simulink library "Tire_Utilities"  (R2026a)
settings: Solver=VariableStepAuto
undefined symbols (not defined in the file or in its folder): X, Y, Z
libraries: simulink x12, nesl_utility x7, sm_lib x7, $bdroot x6
Description:
  | Simscape Vehicle Templates Library
  | 
  | Copyright 2018-2024 The MathWorks, Inc.
settings Model: Creator=smiller  LastModifiedBy=andrei

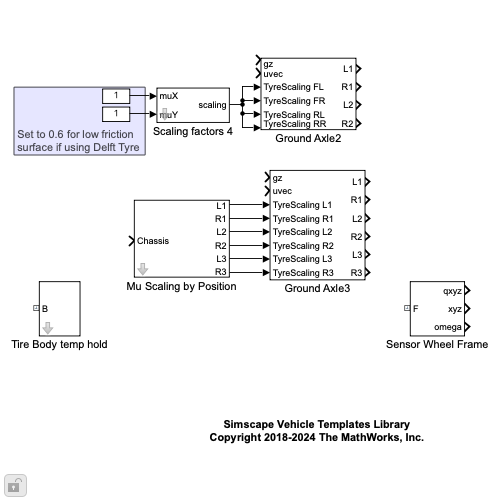
[thumbnail: Simulink's stored preview of the top-level diagram]
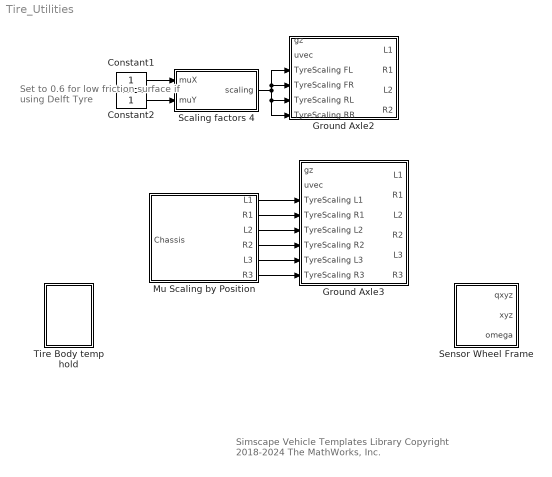
== system Tire_Utilities ==
  note: Set to 0.6 for low friction
      | surface if using Delft Tyre
  note: Simscape Vehicle Templates Library
      | Copyright 2018-2024 The MathWorks, Inc.
  Constant1 : Constant
  Constant2 : Constant
  Ground Axle2 : Subsystem
  Ground Axle3 : Subsystem
  Mu Scaling by Position : Subsystem  mask{muFL_out=1, muFR_out=1, muRL_out=1, muRR_out=1, muFL_in=1, muFR_in=1, muRL_in=1, muRR_in=1, intvX_FL_start=100-40, intvX_FR_start=100-40, intvX_RL_start=100-40, intvX_RR_start=100-40, intvX_FL_end=130-40, intvX_FR_end=130-40, intvX_RL_end=130-40, intvX_RR_end=130-40, intvY_FL_start=-30, intvY_FR_start=-30, intvY_RL_start=-30, intvY_RR_start=-30, intvY_FL_end=0, intvY_FR_end=0, intvY_RL_end=0, intvY_RR_end=0}
      mask TypeOptions muFL_out: muL1 out/Value
      mask TypeOptions muFR_out: muR1 out/Value
      mask TypeOptions muRL_out: muL2 out/Value
      mask TypeOptions muRR_out: muR2 out/Value
      mask TypeOptions muFL_in: muL 1in/Value
      mask TypeOptions muFR_in: muR1 in/Value
      mask TypeOptions muRL_in: muL2 in/Value
      mask TypeOptions muRR_in: muR2 in/Value
      mask TypeOptions intvX_FL_start: Interval Test L1x/lowlimit
      mask TypeOptions intvX_FR_start: Interval Test R1x/lowlimit
      mask TypeOptions intvX_RL_start: Interval Test L2x/lowlimit
      mask TypeOptions intvX_RR_start: Interval Test R2x/lowlimit
      mask TypeOptions intvX_FL_end: Interval Test L1x/uplimit
      mask TypeOptions intvX_FR_end: Interval Test R1x/uplimit
      mask TypeOptions intvX_RL_end: Interval Test L2x/uplimit
      mask TypeOptions intvX_RR_end: Interval Test R2x/uplimit
      mask TypeOptions intvY_FL_start: Interval Test L1y/lowlimit
      mask TypeOptions intvY_FR_start: Interval Test R1y/lowlimit
      mask TypeOptions intvY_RL_start: Interval Test L2y/lowlimit
      mask TypeOptions intvY_RR_start: Interval Test R2y/lowlimit
      mask TypeOptions intvY_FL_end: Interval Test L1y/uplimit
      mask TypeOptions intvY_FR_end: Interval Test R1y/uplimit
      mask TypeOptions intvY_RL_end: Interval Test L2y/uplimit
      mask TypeOptions intvY_RR_end: Interval Test R2y/uplimit
      mask DialogControl text_whl Prompt: Wheel
      mask DialogControl text_FL Prompt: FL
      mask DialogControl text_FR Prompt: FR
      mask DialogControl text_RL Prompt: RL
      mask DialogControl text_RR Prompt: RR
      mask DialogControl text_mu Prompt: mu
      mask DialogControl text_mu_intv Prompt: mu intv
      mask DialogControl text_x_start Prompt: X Start (m)
      mask DialogControl text_x_end Prompt: X End (m)
      mask DialogControl text_y_start Prompt: Y Start (m)
      mask DialogControl text_y_end Prompt: Y End (m)
  Scaling factors 4 : Subsystem  mask{LKX=1, LKY=1, LKYC=1, LTR=1, LKZC=1}
      mask prompts: LKX "longitudinal slip stiffness"; LKY "cornering stiffness"; LKYC "camber stiffness"; LTR "pneumatic trail"; LKZC "camber torque stiffness"
  Sensor Wheel Frame : Subsystem
  Tire Body temp hold : Subsystem  mask{radius=0.4225, rim_radius=0.3048, width=0.235, rim_width=0.235*0.1, mass=10, rim_mass=0, tire_inertia=[1 2], rim_inertia=[0 0], popup_leftRight=Left, clr_tyre=[0.5 0.5 0.5], opc_tyre=1.0, clr_rim=[0.8 0.8 0.8], opc_rim=0.5}
      mask prompts: popup_leftRight "Left/Right"
      mask init:
      | % Change rim location if wheel is on right side
      | if (popup_leftRight == 1)
      |     rhs_tire = 1;
      | elseif(popup_leftRight == 2)
      |     rhs_tire = -1;
      | end
      | 
      | Imat = [tire_inertia(1)+rim_inertia(1) 0 0; 0 tire_inertia(1)+rim_inertia(1) 0; 0 0 tire_inertia(2)+rim_inertia(2)];
      mask TypeOptions popup_leftRight: Left | Right
      mask TypeOptions clr_tyre: Tire/GraphicDiffuseColor
      mask TypeOptions opc_tyre: Tire/GraphicOpacity
      mask TypeOptions clr_rim: Rim/GraphicDiffuseColor
      mask TypeOptions opc_rim: Rim/GraphicOpacity
      mask DialogControl cont_tyre Prompt: Tire Geometry
      mask DialogControl group_tyre_dim Prompt: Dimensions
      mask DialogControl text_tyre_tire Prompt: Tyre
      mask DialogControl text_tyre_rim Prompt: Rim
      mask DialogControl text_tyre_dim_radius Prompt: Radius (m)
      mask DialogControl text_tyre_dim_width Prompt: Width (m)
      mask DialogControl text_tyre_mass Prompt: Mass (kg)
      mask DialogControl text_tyre_inertia Prompt: Inertia [Ixx Iyy]
      mask DialogControl cont_tyre_vis Prompt: Visualization
      mask DialogControl text_vis_tyre_clr Prompt: Color [RGB]
      mask DialogControl text_vis_tyre_opc Prompt: Opacity (0-1)
      mask DialogControl text_vis_tyre_tyre Prompt: Tyre
      mask DialogControl text_vis_tyre_rim Prompt: Rim
  wires:
  Mu Scaling by Position/6(R3) -> Ground Axle3/8(TyreScaling R3)
  Mu Scaling by Position/5(L3) -> Ground Axle3/7(TyreScaling L3)
  Mu Scaling by Position/4(R2) -> Ground Axle3/6(TyreScaling R2)
  Mu Scaling by Position/3(L2) -> Ground Axle3/5(TyreScaling L2)
  Mu Scaling by Position/2(R1) -> Ground Axle3/4(TyreScaling R1)
  Mu Scaling by Position/1(L1) -> Ground Axle3/3(TyreScaling L1)
  Constant2/1 -> Scaling factors 4/2(muY)
  Constant1/1 -> Scaling factors 4/1(muX)
  Scaling factors 4/1(scaling) -> Ground Axle2/4(TyreScaling FR), Ground Axle2/3(TyreScaling FL), Ground Axle2/5(TyreScaling RL), Ground Axle2/6(TyreScaling RR)

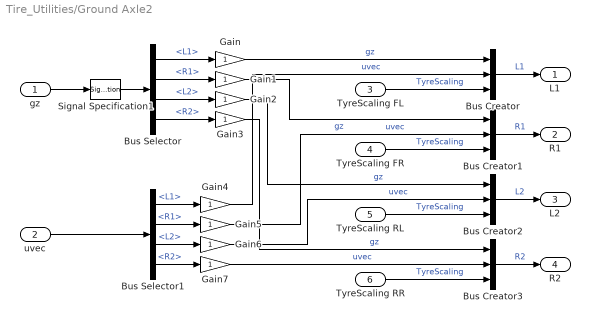
== system Tire_Utilities/Ground Axle2 ==
  gz : Inport
  uvec : Inport  Port=2
  TyreScaling FL : Inport  Port=3
  TyreScaling FR : Inport  Port=4
  TyreScaling RL : Inport  Port=5
  TyreScaling RR : Inport  Port=6
  Bus Creator{,1..3} (4 alike) : BusCreator  Inputs=3
  Bus Selector : BusSelector  OutputSignals=L1,R1,L2,R2
  Bus Selector1 : BusSelector  OutputSignals=L1,R1,L2,R2
  Gain{,1..7} (8 alike) : Gain
  Signal Specification1 : SignalSpecification  Unit=m
  L1 : Outport  VectorParamsAs1DForOutWhenUnconnected=off
  R1 : Outport  Port=2  VectorParamsAs1DForOutWhenUnconnected=off
  L2 : Outport  Port=3  VectorParamsAs1DForOutWhenUnconnected=off
  R2 : Outport  Port=4  VectorParamsAs1DForOutWhenUnconnected=off
  wires:
  Gain7/1 -> Bus Creator3/2  "uvec"
  Gain6/1 -> Bus Creator2/2  "uvec"
  Gain5/1 -> Bus Creator1/2  "uvec"
  Gain4/1 -> Bus Creator/2  "uvec"
  Bus Selector1/4 -> Gain7/1  "<R2>"
  Bus Selector1/3 -> Gain6/1  "<L2>"
  Bus Selector1/2 -> Gain5/1  "<R1>"
  Bus Selector1/1 -> Gain4/1  "<L1>"
  uvec/1 -> Bus Selector1/1
  Bus Selector/4 -> Gain3/1  "<R2>"
  Bus Selector/3 -> Gain2/1  "<L2>"
  Bus Selector/2 -> Gain1/1  "<R1>"
  Gain/1 -> Bus Creator/1  "gz"
  Bus Selector/1 -> Gain/1  "<L1>"
  TyreScaling RR/1 -> Bus Creator3/3  "TyreScaling"
  TyreScaling RL/1 -> Bus Creator2/3  "TyreScaling"
  TyreScaling FR/1 -> Bus Creator1/3  "TyreScaling"
  Gain2/1 -> Bus Creator2/1  "gz"
  Signal Specification1/1 -> Bus Selector/1
  Bus Creator2/1 -> L2/1  "L2"
  Gain3/1 -> Bus Creator3/1  "gz"
  gz/1 -> Signal Specification1/1
  Bus Creator3/1 -> R2/1  "R2"
  TyreScaling FL/1 -> Bus Creator/3  "TyreScaling"
  Gain1/1 -> Bus Creator1/1  "gz"
  Bus Creator1/1 -> R1/1  "R1"
  Bus Creator/1 -> L1/1  "L1"

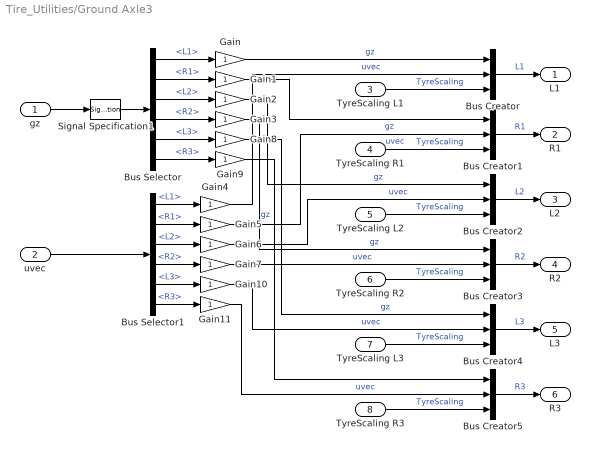
== system Tire_Utilities/Ground Axle3 ==
  gz : Inport
  uvec : Inport  Port=2
  TyreScaling L1 : Inport  Port=3
  TyreScaling R1 : Inport  Port=4
  TyreScaling L2 : Inport  Port=5
  TyreScaling R2 : Inport  Port=6
  TyreScaling L3 : Inport  Port=7
  TyreScaling R3 : Inport  Port=8
  Bus Creator{,1..5} (6 alike) : BusCreator  Inputs=3
  Bus Selector : BusSelector  OutputSignals=L1,R1,L2,R2,L3,R3
  Bus Selector1 : BusSelector  OutputSignals=L1,R1,L2,R2,L3,R3
  Gain{,1..11} (12 alike) : Gain
  Signal Specification1 : SignalSpecification  Unit=m
  L1 : Outport  VectorParamsAs1DForOutWhenUnconnected=off
  R1 : Outport  Port=2  VectorParamsAs1DForOutWhenUnconnected=off
  L2 : Outport  Port=3  VectorParamsAs1DForOutWhenUnconnected=off
  R2 : Outport  Port=4  VectorParamsAs1DForOutWhenUnconnected=off
  L3 : Outport  Port=5  VectorParamsAs1DForOutWhenUnconnected=off
  R3 : Outport  Port=6  VectorParamsAs1DForOutWhenUnconnected=off
  wires:
  Bus Selector/6 -> Gain9/1  "<R3>"
  Bus Selector/5 -> Gain8/1  "<L3>"
  Bus Selector1/6 -> Gain11/1  "<R3>"
  Bus Selector1/5 -> Gain10/1  "<L3>"
  Gain11/1 -> Bus Creator5/2  "uvec"
  Gain10/1 -> Bus Creator4/2  "uvec"
  TyreScaling R3/1 -> Bus Creator5/3  "TyreScaling"
  TyreScaling L3/1 -> Bus Creator4/3  "TyreScaling"
  Gain8/1 -> Bus Creator4/1  "gz"
  Bus Creator4/1 -> L3/1  "L3"
  Gain9/1 -> Bus Creator5/1  "gz"
  Bus Creator5/1 -> R3/1  "R3"
  Bus Creator/1 -> L1/1  "L1"
  Bus Creator1/1 -> R1/1  "R1"
  Gain1/1 -> Bus Creator1/1  "gz"
  TyreScaling L1/1 -> Bus Creator/3  "TyreScaling"
  Bus Creator3/1 -> R2/1  "R2"
  gz/1 -> Signal Specification1/1
  Gain3/1 -> Bus Creator3/1  "gz"
  Bus Creator2/1 -> L2/1  "L2"
  Signal Specification1/1 -> Bus Selector/1
  Gain2/1 -> Bus Creator2/1  "gz"
  TyreScaling R1/1 -> Bus Creator1/3  "TyreScaling"
  TyreScaling L2/1 -> Bus Creator2/3  "TyreScaling"
  TyreScaling R2/1 -> Bus Creator3/3  "TyreScaling"
  Bus Selector/1 -> Gain/1  "<L1>"
  Gain/1 -> Bus Creator/1  "gz"
  Bus Selector/2 -> Gain1/1  "<R1>"
  Bus Selector/3 -> Gain2/1  "<L2>"
  Bus Selector/4 -> Gain3/1  "<R2>"
  uvec/1 -> Bus Selector1/1
  Bus Selector1/1 -> Gain4/1  "<L1>"
  Bus Selector1/2 -> Gain5/1  "<R1>"
  Bus Selector1/3 -> Gain6/1  "<L2>"
  Bus Selector1/4 -> Gain7/1  "<R2>"
  Gain4/1 -> Bus Creator/2  "uvec"
  Gain5/1 -> Bus Creator1/2  "uvec"
  Gain6/1 -> Bus Creator2/2  "uvec"
  Gain7/1 -> Bus Creator3/2  "uvec"

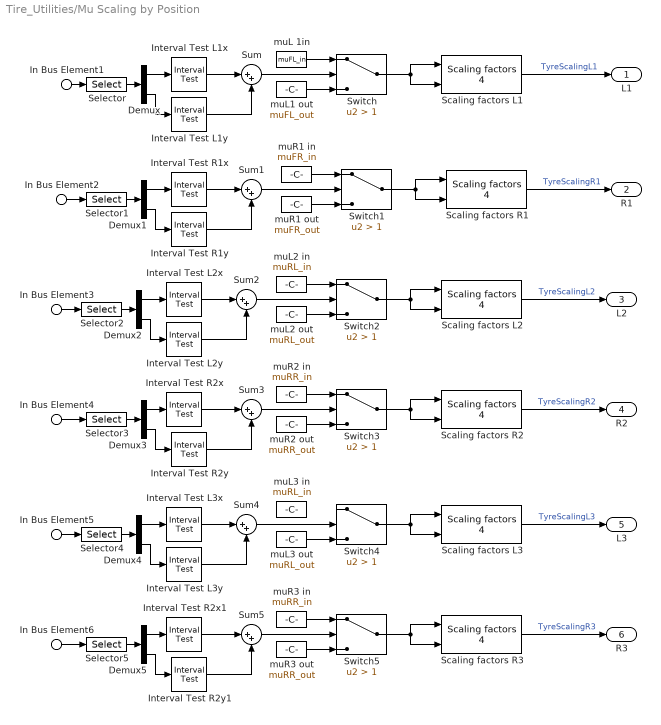
== system Tire_Utilities/Mu Scaling by Position ==
  In Bus Element1 : Inport  PortName=Chassis  Element=WhlL1.xyz
  In Bus Element2 : Inport  PortName=Chassis  Element=WhlR1.xyz
  In Bus Element3 : Inport  PortName=Chassis  Element=WhlL2.xyz
  In Bus Element4 : Inport  PortName=Chassis  Element=WhlR2.xyz
  In Bus Element5 : Inport  PortName=Chassis  Element=WhlL3.xyz
  In Bus Element6 : Inport  PortName=Chassis  Element=WhlR3.xyz
  Demux{,1..5} (6 alike) : Demux  Outputs=2
  Interval Test L1x : simulink/Logic and Bit Operations/Interval Test  IntervalClosedRight=on  uplimit=intvX_FL_end  IntervalClosedLeft=on  lowlimit=intvX_FL_start  OutDataTypeStr=uint8
  Interval Test L1y : simulink/Logic and Bit Operations/Interval Test  IntervalClosedRight=on  uplimit=intvY_FL_end  IntervalClosedLeft=on  lowlimit=intvY_FL_start  OutDataTypeStr=uint8
  Interval Test L2x : simulink/Logic and Bit Operations/Interval Test  IntervalClosedRight=on  uplimit=intvX_RL_end  IntervalClosedLeft=on  lowlimit=intvX_RL_start  OutDataTypeStr=uint8
  Interval Test L2y : simulink/Logic and Bit Operations/Interval Test  IntervalClosedRight=on  uplimit=intvY_RL_end  IntervalClosedLeft=on  lowlimit=intvY_RL_start  OutDataTypeStr=uint8
  Interval Test L3x : simulink/Logic and Bit Operations/Interval Test  IntervalClosedRight=on  uplimit=intvX_RL_end  IntervalClosedLeft=on  lowlimit=intvX_RL_start  OutDataTypeStr=uint8
  Interval Test L3y : simulink/Logic and Bit Operations/Interval Test  IntervalClosedRight=on  uplimit=intvY_RL_end  IntervalClosedLeft=on  lowlimit=intvY_RL_start  OutDataTypeStr=uint8
  Interval Test R1x : simulink/Logic and Bit Operations/Interval Test  IntervalClosedRight=on  uplimit=intvX_FR_end  IntervalClosedLeft=on  lowlimit=intvX_FR_start  OutDataTypeStr=uint8
  Interval Test R1y : simulink/Logic and Bit Operations/Interval Test  IntervalClosedRight=on  uplimit=intvY_FR_end  IntervalClosedLeft=on  lowlimit=intvY_FR_start  OutDataTypeStr=uint8
  Interval Test R2x : simulink/Logic and Bit Operations/Interval Test  IntervalClosedRight=on  uplimit=intvX_RR_end  IntervalClosedLeft=on  lowlimit=intvX_RR_start  OutDataTypeStr=uint8
  Interval Test R2x1 : simulink/Logic and Bit Operations/Interval Test  IntervalClosedRight=on  uplimit=intvX_RR_end  IntervalClosedLeft=on  lowlimit=intvX_RR_start  OutDataTypeStr=uint8
  Interval Test R2y : simulink/Logic and Bit Operations/Interval Test  IntervalClosedRight=on  uplimit=intvY_RR_end  IntervalClosedLeft=on  lowlimit=intvY_RR_start  OutDataTypeStr=uint8
  Interval Test R2y1 : simulink/Logic and Bit Operations/Interval Test  IntervalClosedRight=on  uplimit=intvY_RR_end  IntervalClosedLeft=on  lowlimit=intvY_RR_start  OutDataTypeStr=uint8
  Scaling factors L1 : $bdroot/Scaling factors 4  LKX=1  LKY=1  LKYC=1  LTR=1  LKZC=1
  Scaling factors L2 : $bdroot/Scaling factors 4  LKX=1  LKY=1  LKYC=1  LTR=1  LKZC=1
  Scaling factors L3 : $bdroot/Scaling factors 4  LKX=1  LKY=1  LKYC=1  LTR=1  LKZC=1
  Scaling factors R1 : $bdroot/Scaling factors 4  LKX=1  LKY=1  LKYC=1  LTR=1  LKZC=1
  Scaling factors R2 : $bdroot/Scaling factors 4  LKX=1  LKY=1  LKYC=1  LTR=1  LKZC=1
  Scaling factors R3 : $bdroot/Scaling factors 4  LKX=1  LKY=1  LKYC=1  LTR=1  LKZC=1
  Selector{,1..5} (6 alike) : Selector  InputPortWidth=3  IndexOptions=Index vector (dialog)  Indices=[1 2]  OutputSizes=1
  Sum{,1..5} (6 alike) : Sum  Inputs=|++
  Switch : Switch  Criteria=u2 > Threshold  Threshold=1  ZeroCross=off  SaturateOnIntegerOverflow=off  InputSameDT=off
  Switch{1..5} (5 alike) : Switch  Criteria=u2 > Threshold  Threshold=1  SaturateOnIntegerOverflow=off  InputSameDT=off
  muL 1in : Constant  Value=muFL_in
  muL1 out : Constant  Value=muFL_out
  muL2 in : Constant  Value=muRL_in
  muL2 out : Constant  Value=muRL_out
  muL3 in : Constant  Value=muRL_in
  muL3 out : Constant  Value=muRL_out
  muR1 in : Constant  Value=muFR_in
  muR1 out : Constant  Value=muFR_out
  muR2 in : Constant  Value=muRR_in
  muR2 out : Constant  Value=muRR_out
  muR3 in : Constant  Value=muRR_in
  muR3 out : Constant  Value=muRR_out
  L1 : Outport  VectorParamsAs1DForOutWhenUnconnected=off
  R1 : Outport  Port=2  VectorParamsAs1DForOutWhenUnconnected=off
  L2 : Outport  Port=3  VectorParamsAs1DForOutWhenUnconnected=off
  R2 : Outport  Port=4  VectorParamsAs1DForOutWhenUnconnected=off
  L3 : Outport  Port=5  VectorParamsAs1DForOutWhenUnconnected=off
  R3 : Outport  Port=6  VectorParamsAs1DForOutWhenUnconnected=off
  wires:
  Interval Test R2x1/1 -> Sum5/1
  Demux5/2 -> Interval Test R2y1/1
  Demux5/1 -> Interval Test R2x1/1
  Sum5/1 -> Switch5/2
  Selector5/1 -> Demux5/1
  In Bus Element6/1 -> Selector5/1
  Interval Test R2y1/1 -> Sum5/2
  Demux4/2 -> Interval Test L3y/1
  Selector4/1 -> Demux4/1
  Demux4/1 -> Interval Test L3x/1
  Interval Test L3y/1 -> Sum4/2
  Sum4/1 -> Switch4/2
  In Bus Element5/1 -> Selector4/1
  Interval Test L3x/1 -> Sum4/1
  muR3 out/1 -> Switch5/3
  muR3 in/1 -> Switch5/1
  Switch5/1 -> Scaling factors R3/2, Scaling factors R3/1
  Scaling factors R3/1 -> R3/1  "TyreScalingR3"
  Scaling factors L3/1 -> L3/1  "TyreScalingL3"
  Switch4/1 -> Scaling factors L3/1, Scaling factors L3/2
  muL3 out/1 -> Switch4/3
  In Bus Element1/1 -> Selector/1
  muL 1in/1 -> Switch/1
  muL1 out/1 -> Switch/3
  Switch/1 -> Scaling factors L1/2, Scaling factors L1/1
  Scaling factors L1/1 -> L1/1  "TyreScalingL1"
  Scaling factors R1/1 -> R1/1  "TyreScalingR1"
  Switch1/1 -> Scaling factors R1/1, Scaling factors R1/2
  muR1 in/1 -> Switch1/1
  In Bus Element2/1 -> Selector1/1
  muR1 out/1 -> Switch1/3
  muL2 out/1 -> Switch2/3
  muL2 in/1 -> Switch2/1
  Switch2/1 -> Scaling factors L2/2, Scaling factors L2/1
  Scaling factors L2/1 -> L2/1  "TyreScalingL2"
  Scaling factors R2/1 -> R2/1  "TyreScalingR2"
  Switch3/1 -> Scaling factors R2/1, Scaling factors R2/2
  muR2 in/1 -> Switch3/1
  muR2 out/1 -> Switch3/3
  Selector/1 -> Demux/1
  Demux/2 -> Interval Test L1y/1
  Sum/1 -> Switch/2
  Interval Test L1y/1 -> Sum/2
  Interval Test L1x/1 -> Sum/1
  Interval Test R1x/1 -> Sum1/1
  Demux1/1 -> Interval Test R1x/1
  Sum1/1 -> Switch1/2
  Demux1/2 -> Interval Test R1y/1
  Selector1/1 -> Demux1/1
  Interval Test R1y/1 -> Sum1/2
  Interval Test L2x/1 -> Sum2/1
  In Bus Element3/1 -> Selector2/1
  Sum2/1 -> Switch2/2
  Interval Test L2y/1 -> Sum2/2
  Demux2/1 -> Interval Test L2x/1
  Selector2/1 -> Demux2/1
  Demux2/2 -> Interval Test L2y/1
  Interval Test R2y/1 -> Sum3/2
  In Bus Element4/1 -> Selector3/1
  Selector3/1 -> Demux3/1
  Sum3/1 -> Switch3/2
  Demux3/1 -> Interval Test R2x/1
  Demux3/2 -> Interval Test R2y/1
  Interval Test R2x/1 -> Sum3/1
  Demux/1 -> Interval Test L1x/1

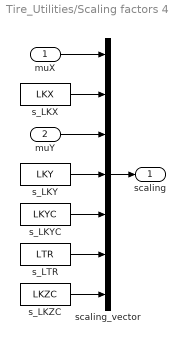
== system Tire_Utilities/Scaling factors 4 ==
  muX : Inport
  muY : Inport  Port=2
  s_LKX : Constant  Value=LKX
  s_LKY : Constant  Value=LKY
  s_LKYC : Constant  Value=LKYC
  s_LKZC : Constant  Value=LKZC
  s_LTR : Constant  Value=LTR
  scaling_vector : Mux  Inputs=7
  scaling : Outport  VectorParamsAs1DForOutWhenUnconnected=off
  wires:
  scaling_vector/1 -> scaling/1
  s_LKZC/1 -> scaling_vector/7
  s_LTR/1 -> scaling_vector/6
  s_LKYC/1 -> scaling_vector/5
  s_LKY/1 -> scaling_vector/4
  muY/1 -> scaling_vector/3
  s_LKX/1 -> scaling_vector/2
  muX/1 -> scaling_vector/1

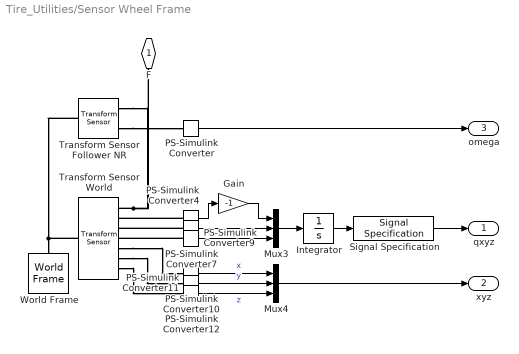
== system Tire_Utilities/Sensor Wheel Frame ==
  Gain : Gain  Gain=-1
  Integrator : Integrator  WrappedStateUpperValue=2*pi  WrappedStateLowerValue=0
  Mux3 : Mux  Inputs=3
  Mux4 : Mux  Inputs=3
  PS-Simulink Converter{,4,7,9} (4 alike) : nesl_utility/PS-Simulink Converter  PhysicalDomain=network_engine_domain  SubClassName=ps_output  LeftPortType=input  RightPortType=output  PseudoPeriodic=off  Frequencies=[]  VectorFormat=1-D array  Unit=rad/s  AffineConversion=off
  PS-Simulink Converter10 : nesl_utility/PS-Simulink Converter  PhysicalDomain=network_engine_domain  SubClassName=ps_output  LeftPortType=input  RightPortType=output  PseudoPeriodic=off  Frequencies=[]  VectorFormat=1-D array  Unit=m  AffineConversion=off
  PS-Simulink Converter11 : nesl_utility/PS-Simulink Converter  PhysicalDomain=network_engine_domain  SubClassName=ps_output  LeftPortType=input  RightPortType=output  PseudoPeriodic=off  Frequencies=[]  VectorFormat=1-D array  Unit=m  AffineConversion=off
  PS-Simulink Converter12 : nesl_utility/PS-Simulink Converter  PhysicalDomain=network_engine_domain  SubClassName=ps_output  LeftPortType=input  RightPortType=output  PseudoPeriodic=off  Frequencies=[]  VectorFormat=1-D array  Unit=m  AffineConversion=off
  Signal Specification : SignalSpecification  Unit=rad
  Transform Sensor Follower NR : sm_lib/Frames and Transforms/Transform Sensor  MeasurementFrame=NonRotatingFollower  RotationSequence=XYX  SenseAngle=off  SenseAxis=off  SenseQ=off  SenseR=off  SenseRotationSequence=off  SenseOmegaX=off  SenseOmegaY=off  SenseOmegaZ=on  SenseOmega=off  SenseQDot=off  SenseRDot=off  SenseRotationSequenceDot=off  SenseAlphaX=off  SenseAlphaY=off  SenseAlphaZ=off  SenseAlpha=off  SenseQDDot=off  SenseRDDot=off  SenseX=off  SenseY=off  SenseZ=off  SenseXYZ=off  SenseRad=off  SenseAzim=off  SenseDist=off  SenseInc=off  SenseXDot=off  SenseYDot=off  SenseZDot=off  SenseXYZDot=off  SenseRadDot=off  SenseAzimDot=off  SenseDistDot=off  SenseIncDot=off  SenseXDDot=off  SenseYDDot=off  SenseZDDot=off  SenseXYZDDot=off  SenseRadDDot=off  SenseAzimDDot=off  SenseDistDDot=off  SenseIncDDot=off
  Transform Sensor World : sm_lib/Frames and Transforms/Transform Sensor  MeasurementFrame=World  RotationSequence=XYX  SenseAngle=off  SenseAxis=off  SenseQ=off  SenseR=off  SenseRotationSequence=off  SenseOmegaX=on  SenseOmegaY=on  SenseOmegaZ=on  SenseOmega=off  SenseQDot=off  SenseRDot=off  SenseRotationSequenceDot=off  SenseAlphaX=off  SenseAlphaY=off  SenseAlphaZ=off  SenseAlpha=off  SenseQDDot=off  SenseRDDot=off  SenseX=on  SenseY=on  SenseZ=on  SenseXYZ=off  SenseRad=off  SenseAzim=off  SenseDist=off  SenseInc=off  SenseXDot=off  SenseYDot=off  SenseZDot=off  SenseXYZDot=off  SenseRadDot=off  SenseAzimDot=off  SenseDistDot=off  SenseIncDot=off  SenseXDDot=off  SenseYDDot=off  SenseZDDot=off  SenseXYZDDot=off  SenseRadDDot=off  SenseAzimDDot=off  SenseDistDDot=off  SenseIncDDot=off
  World Frame : sm_lib/Frames and Transforms/World Frame
  F : PMIOPort  Side=Left
  qxyz : Outport  VectorParamsAs1DForOutWhenUnconnected=off
  xyz : Outport  Port=2  VectorParamsAs1DForOutWhenUnconnected=off
  omega : Outport  Port=3  VectorParamsAs1DForOutWhenUnconnected=off
  wires:
  Signal Specification/1 -> qxyz/1
  PS-Simulink Converter/1 -> omega/1
  Mux4/1 -> xyz/1
  Integrator/1 -> Signal Specification/1
  PS-Simulink Converter4/1 -> Gain/1
  PS-Simulink Converter9/1 -> Mux3/3
  PS-Simulink Converter11/1 -> Mux4/2  "y"
  PS-Simulink Converter10/1 -> Mux4/1  "x"
  PS-Simulink Converter12/1 -> Mux4/3  "z"
  Gain/1 -> Mux3/1
  PS-Simulink Converter7/1 -> Mux3/2
  Mux3/1 -> Integrator/1
  connections:
  Transform Sensor Follower NR/RConn2 -- PS-Simulink Converter/LConn1
  Transform Sensor World/RConn5 -- PS-Simulink Converter10/LConn1
  Transform Sensor World/RConn7 -- PS-Simulink Converter12/LConn1
  PS-Simulink Converter4/LConn1 -- Transform Sensor World/RConn2
  Transform Sensor World/RConn1 -- F/RConn1 -- Transform Sensor Follower NR/RConn1
  PS-Simulink Converter9/LConn1 -- Transform Sensor World/RConn4
  World Frame/RConn1 -- Transform Sensor Follower NR/LConn1 -- Transform Sensor World/LConn1
  PS-Simulink Converter7/LConn1 -- Transform Sensor World/RConn3
  Transform Sensor World/RConn6 -- PS-Simulink Converter11/LConn1

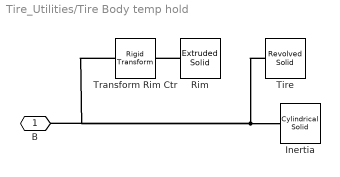
== system Tire_Utilities/Tire Body temp hold ==
  Inertia : sm_lib/Body Elements/Cylindrical Solid  CylinderRadius=0.001  CylinderRadiusUnits=m  CylinderLength=0.001  CylinderLengthUnits=m  ExportEntireGeometry=off  InertiaType=Custom  BasedOnType=Density  Density=1000  DensityUnits=kg/(m^3)  Mass=mass  MassUnits=kg  CenterOfMass=[0 0 0]  CenterOfMassUnits=m  MomentsOfInertia=[Imat(1,1) Imat(2,2) Imat(3,3)]  MomentsOfInertiaUnits=kg*m^2  ProductsOfInertia=[0 0 0]  ProductsOfInertiaUnits=kg*m^2  GraphicType=FromGeometry  MarkerShape=Sphere  MarkerSize=10  GraphicVisPropType=SimpleVisualProperties  GraphicDiffuseColor=[0.2 0.8 1.0]  GraphicOpacity=1.0  GraphicSpecularColor=[0.5 0.5 0.5 1.0]  GraphicAmbientColor=[0.15 0.15 0.15 1.0]  GraphicEmissiveColor=[0.0 0.0 0.0 1.0]  GraphicShininess=75  DoExposeReferenceFrame=on  SerializedFrames=<Frames/>
  Rim : sm_lib/Body Elements/Extruded Solid  ExtrusionType=Regular  PolygonNumSides=5  PolygonOuterRadius=rim_radius  PolygonOuterRadiusUnits=m  ExportEntireGeometry=off  ExtrusionCrossSection=[1 1; -1 1; -1 -1; 1 -1]  ExtrusionCrossSectionUnits=m  ExportConvexHullGeometry=off  ExtrusionLength=width*0.1  ExtrusionLengthUnits=m  InertiaType=Custom  BasedOnType=Density  Density=1000  DensityUnits=kg/(m^3)  Mass=0  MassUnits=kg  CenterOfMass=[0 0 0]  CenterOfMassUnits=m  MomentsOfInertia=[0 0 0]  MomentsOfInertiaUnits=kg*m^2  ProductsOfInertia=[0 0 0]  ProductsOfInertiaUnits=kg*m^2  GraphicType=FromGeometry  MarkerShape=Sphere  MarkerSize=10  GraphicVisPropType=SimpleVisualProperties  GraphicDiffuseColor=clr_rim  GraphicOpacity=opc_rim  GraphicSpecularColor=[0.5 0.5 0.5 1.0]  GraphicAmbientColor=[0.15 0.15 0.15 1.0]  GraphicEmissiveColor=[0.0 0.0 0.0 1.0]  GraphicShininess=75  DoExposeReferenceFrame=on  SerializedFrames=<Frames/>
  Tire : sm_lib/Body Elements/Revolved Solid  RevolutionCrossSection="[1  0.5; rim_radius/radius 0.5; rim_radius/radius -0.5; 1 -0.5].*[radius  width]"  RevolutionCrossSectionUnits=m  RevolutionExtent=Full  RevolutionAngle=180  RevolutionAngleUnits=deg  ExportConvexHullGeometry=off  InertiaType=Custom  BasedOnType=Density  Density=1000  DensityUnits=kg/(m^3)  Mass=0  MassUnits=kg  CenterOfMass=[0 0 0]  CenterOfMassUnits=m  MomentsOfInertia=[0 0 0]  MomentsOfInertiaUnits=kg*m^2  ProductsOfInertia=[0 0 0]  ProductsOfInertiaUnits=kg*m^2  GraphicType=FromGeometry  MarkerShape=Sphere  MarkerSize=10  GraphicVisPropType=SimpleVisualProperties  GraphicDiffuseColor=clr_tyre  GraphicOpacity=opc_tyre  GraphicSpecularColor=[0.5 0.5 0.5 1.0]  GraphicAmbientColor=[0.15 0.15 0.15 1.0]  GraphicEmissiveColor=[0.0 0.0 0.0 1.0]  GraphicShininess=75  DoExposeReferenceFrame=on  SerializedFrames=<Frames/>
  Transform Rim Ctr : sm_lib/Frames and Transforms/Rigid Transform  RotationMethod=None  FollAlignAxisA=+X  BaseAlignAxisA=+Y  FollAlignAxisB=+Y  BaseAlignAxisB=+Z  RotationStandardAxis=+Z  RotationAngle=0.0  RotationAngleUnits=deg  RotationArbitraryAxis=[0 0 1]  RotationSequenceAxes=FollowerAxes  RotationSequence=XYX  RotationSequenceAngles=[0 0 0]  RotationSequenceAnglesUnits=deg  RotationMatrix=[1 0 0; 0 1 0; 0 0 1]  Quaternion=[1 0 0 0]  TranslationMethod=StandardAxis  TranslationCartesianOffset=[0 0 0]  TranslationCartesianOffsetUnits=m  TranslationStandardAxis=+Z  TranslationStandardOffset=width*0.4*rhs_tire  TranslationStandardOffsetUnits=m  TranslationROffset=0  TranslationROffsetUnits=m  TranslationThetaOffset=0  TranslationThetaOffsetUnits=deg  TranslationZOffset=0  TranslationZOffsetUnits=m
  B : PMIOPort  Side=Left
  connections:
  Tire/RConn1 -- Inertia/RConn1 -- Transform Rim Ctr/LConn1 -- B/RConn1
  Rim/RConn1 -- Transform Rim Ctr/RConn1
